simulink model "three_phase_power_meter_iec"  (R2026a)
settings: Solver=VariableStepAuto
undefined symbols (not defined in the file): glb_time, grid_emu, magnitude
libraries: simulink x12
(part 1 of 3)
settings Model: Creator=dbagn  LastModifiedBy=dbagn

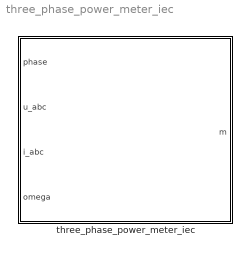
== system three_phase_power_meter_iec ==
  three_phase_power_meter_iec : Subsystem  mask{period=pi/grid_emu.omega_grid_nom, ts=glb_time.ts_afe, enable_time=0.025}
      mask prompts: period "period (s)"; ts "sampling time (s)"; enable_time "enable_time (s)"

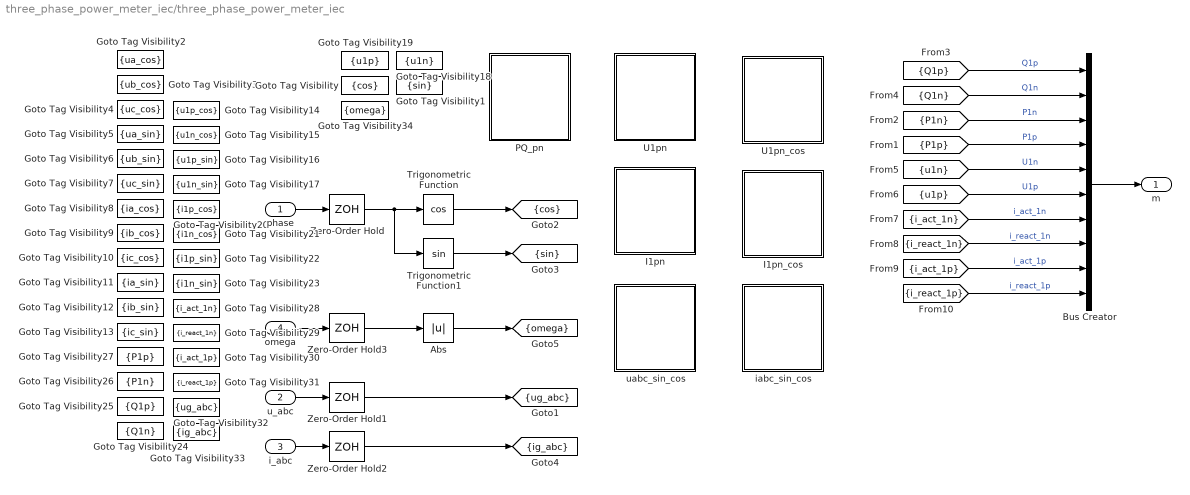
== system three_phase_power_meter_iec/three_phase_power_meter_iec ==
  phase : Inport
  u_abc : Inport  Port=2
  i_abc : Inport  Port=3
  omega : Inport  Port=4
  Abs : Abs  SaturateOnIntegerOverflow=off
  Bus Creator : BusCreator  Inputs=10
  Goto Tag Visibility : GotoTagVisibility  GotoTag=cos
  Goto Tag Visibility1 : GotoTagVisibility  GotoTag=sin
  Goto Tag Visibility10 : GotoTagVisibility  GotoTag=ic_cos
  Goto Tag Visibility11 : GotoTagVisibility  GotoTag=ia_sin
  Goto Tag Visibility12 : GotoTagVisibility  GotoTag=ib_sin
  Goto Tag Visibility13 : GotoTagVisibility  GotoTag=ic_sin
  Goto Tag Visibility14 : GotoTagVisibility  GotoTag=u1p_cos
  Goto Tag Visibility15 : GotoTagVisibility  GotoTag=u1n_cos
  Goto Tag Visibility16 : GotoTagVisibility  GotoTag=u1p_sin
  Goto Tag Visibility17 : GotoTagVisibility  GotoTag=u1n_sin
  Goto Tag Visibility18 : GotoTagVisibility  GotoTag=u1n
  Goto Tag Visibility19 : GotoTagVisibility  GotoTag=u1p
  Goto Tag Visibility2 : GotoTagVisibility  GotoTag=ua_cos
  Goto Tag Visibility20 : GotoTagVisibility  GotoTag=i1p_cos
  Goto Tag Visibility21 : GotoTagVisibility  GotoTag=i1n_cos
  Goto Tag Visibility22 : GotoTagVisibility  GotoTag=i1p_sin
  Goto Tag Visibility23 : GotoTagVisibility  GotoTag=i1n_sin
  Goto Tag Visibility24 : GotoTagVisibility  GotoTag=Q1n
  Goto Tag Visibility25 : GotoTagVisibility  GotoTag=Q1p
  Goto Tag Visibility26 : GotoTagVisibility  GotoTag=P1n
  Goto Tag Visibility27 : GotoTagVisibility  GotoTag=P1p
  Goto Tag Visibility28 : GotoTagVisibility  GotoTag=i_act_1n
  Goto Tag Visibility29 : GotoTagVisibility  GotoTag=i_react_1n
  Goto Tag Visibility3 : GotoTagVisibility  GotoTag=ub_cos
  Goto Tag Visibility30 : GotoTagVisibility  GotoTag=i_act_1p
  Goto Tag Visibility31 : GotoTagVisibility  GotoTag=i_react_1p
  Goto Tag Visibility32 : GotoTagVisibility  GotoTag=ug_abc
  Goto Tag Visibility33 : GotoTagVisibility  GotoTag=ig_abc
  Goto Tag Visibility34 : GotoTagVisibility  GotoTag=omega
  Goto Tag Visibility4 : GotoTagVisibility  GotoTag=uc_cos
  Goto Tag Visibility5 : GotoTagVisibility  GotoTag=ua_sin
  Goto Tag Visibility6 : GotoTagVisibility  GotoTag=ub_sin
  Goto Tag Visibility7 : GotoTagVisibility  GotoTag=uc_sin
  Goto Tag Visibility8 : GotoTagVisibility  GotoTag=ia_cos
  Goto Tag Visibility9 : GotoTagVisibility  GotoTag=ib_cos
  I1pn : Subsystem
  I1pn_cos : Subsystem
  PQ_pn : Subsystem
  Trigonometric Function : Trigonometry  Operator=cos
  Trigonometric Function1 : Trigonometry
  U1pn : Subsystem
  U1pn_cos : Subsystem
  Zero-Order Hold{,1..3} (4 alike) : ZeroOrderHold  SampleTime=ts
  iabc_sin_cos : Subsystem
  uabc_sin_cos : Subsystem
  m : Outport
  tag scope: cos=scoped, ig_abc=scoped, omega=scoped, sin=scoped, ug_abc=scoped
  wires:
  Abs/1 -> [omega]
  [Q1p] -> Bus Creator/1  "Q1p"
  [Q1n] -> Bus Creator/2  "Q1n"
  [P1n] -> Bus Creator/3  "P1n"
  [P1p] -> Bus Creator/4  "P1p"
  Zero-Order Hold3/1 -> Abs/1
  omega/1 -> Zero-Order Hold3/1
  Zero-Order Hold1/1 -> [ug_abc]
  Zero-Order Hold2/1 -> [ig_abc]
  Zero-Order Hold/1 -> Trigonometric Function1/1, Trigonometric Function/1
  Bus Creator/1 -> m/1
  i_abc/1 -> Zero-Order Hold2/1
  u_abc/1 -> Zero-Order Hold1/1
  [i_react_1p] -> Bus Creator/10  "i_react_1p"
  [i_act_1p] -> Bus Creator/9  "i_act_1p"
  [i_react_1n] -> Bus Creator/8  "i_react_1n"
  [i_act_1n] -> Bus Creator/7  "i_act_1n"
  [u1p] -> Bus Creator/6  "U1p"
  [u1n] -> Bus Creator/5  "U1n"
  phase/1 -> Zero-Order Hold/1
  Trigonometric Function/1 -> [cos]
  Trigonometric Function1/1 -> [sin]

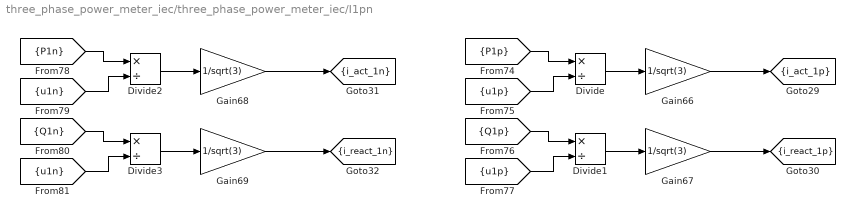
== system three_phase_power_meter_iec/three_phase_power_meter_iec/I1pn ==
  Divide{,1..3} (4 alike) : Product  Inputs=*/
  Gain{66..69} (4 alike) : Gain  Gain=1/sqrt(3)
  tag scope: i_act_1n=scoped, i_act_1p=scoped, i_react_1n=scoped, i_react_1p=scoped
  wires:
  [P1n] -> Divide2/1
  [Q1n] -> Divide3/1
  [u1n] -> Divide3/2
  [Q1p] -> Divide1/1
  Gain69/1 -> [i_react_1n]
  [u1p] -> Divide/2
  Divide/1 -> Gain66/1
  Divide3/1 -> Gain69/1
  Divide1/1 -> Gain67/1
  Gain66/1 -> [i_act_1p]
  [u1n] -> Divide2/2
  Gain67/1 -> [i_react_1p]
  [u1p] -> Divide1/2
  Gain68/1 -> [i_act_1n]
  Divide2/1 -> Gain68/1
  [P1p] -> Divide/1

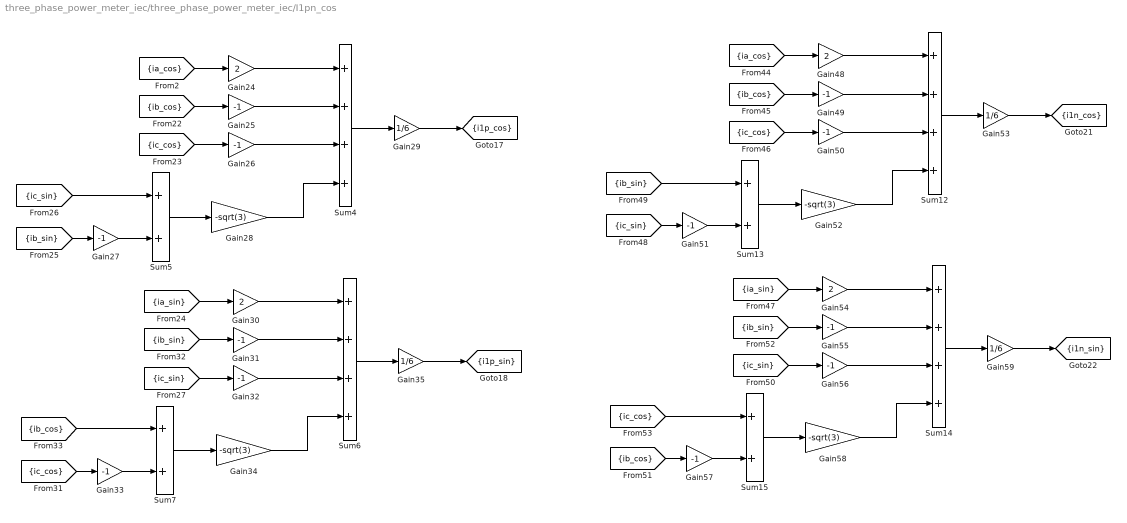
== system three_phase_power_meter_iec/three_phase_power_meter_iec/I1pn_cos ==
  Gain{24,30,48,54} (4 alike) : Gain  Gain=2
  Gain{25..27,31..33,49..51,55..57} (12 alike) : Gain  Gain=-1
  Gain{28,34,52,58} (4 alike) : Gain  Gain=-sqrt(3)
  Gain{29,35,53,59} (4 alike) : Gain  Gain=1/6
  Sum{4,6,12,14} (4 alike) : Sum  Inputs=++++
  Sum{5,7,13,15} (4 alike) : Sum
  tag scope: i1n_cos=scoped, i1n_sin=scoped, i1p_cos=scoped, i1p_sin=scoped
  wires:
  Gain57/1 -> Sum15/2
  [ib_cos] -> Gain25/1
  Sum15/1 -> Gain58/1
  Gain50/1 -> Sum12/3
  [ib_sin] -> Gain31/1
  Gain56/1 -> Sum14/3
  [ic_cos] -> Gain50/1
  Gain48/1 -> Sum12/1
  [ia_sin] -> Gain30/1
  Gain51/1 -> Sum13/2
  Sum6/1 -> Gain35/1
  Gain59/1 -> [i1n_sin]
  Gain58/1 -> Sum14/4
  Gain26/1 -> Sum4/3
  [ib_sin] -> Gain55/1
  Gain32/1 -> Sum6/3
  Gain28/1 -> Sum4/4
  [ia_cos] -> Gain24/1
  Gain34/1 -> Sum6/4
  [ic_cos] -> Sum15/1
  [ib_cos] -> Gain57/1
  Gain33/1 -> Sum7/2
  Sum5/1 -> Gain28/1
  Sum7/1 -> Gain34/1
  Gain53/1 -> [i1n_cos]
  [ib_sin] -> Gain27/1
  Gain25/1 -> Sum4/2
  [ic_sin] -> Gain56/1
  [ib_sin] -> Sum13/1
  [ib_cos] -> Gain49/1
  Gain24/1 -> Sum4/1
  Sum4/1 -> Gain29/1
  Sum13/1 -> Gain52/1
  [ia_sin] -> Gain54/1
  [ia_cos] -> Gain48/1
  [ic_cos] -> Gain26/1
  Gain30/1 -> Sum6/1
  [ic_sin] -> Sum5/1
  Gain55/1 -> Sum14/2
  [ic_cos] -> Gain33/1
  [ic_sin] -> Gain32/1
  Gain29/1 -> [i1p_cos]
  [ic_sin] -> Gain51/1
  Sum14/1 -> Gain59/1
  Gain31/1 -> Sum6/2
  Gain52/1 -> Sum12/4
  [ib_cos] -> Sum7/1
  Gain54/1 -> Sum14/1
  Gain49/1 -> Sum12/2
  Gain27/1 -> Sum5/2
  Sum12/1 -> Gain53/1
  Gain35/1 -> [i1p_sin]

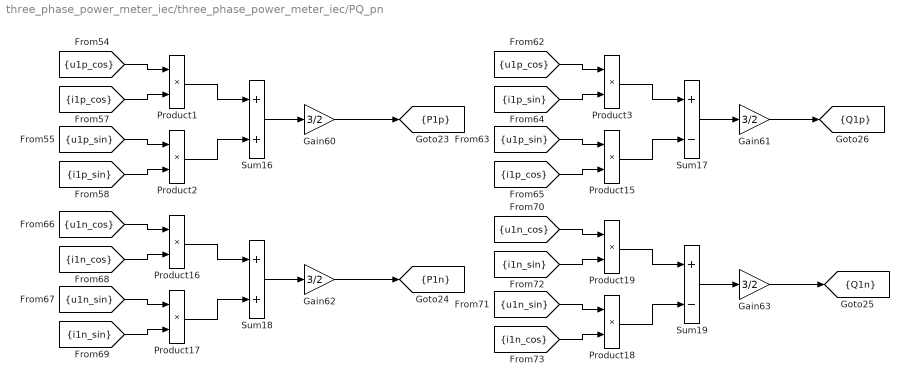
== system three_phase_power_meter_iec/three_phase_power_meter_iec/PQ_pn ==
  Gain{60..63} (4 alike) : Gain  Gain=3/2
  Product{1..3,15..19} (8 alike) : Product  RndMeth=Zero
  Sum16 : Sum
  Sum17 : Sum  Inputs=+-
  Sum18 : Sum
  Sum19 : Sum  Inputs=+-
  tag scope: P1n=scoped, P1p=scoped, Q1n=scoped, Q1p=scoped
  wires:
  Product3/1 -> Sum17/1
  [i1n_sin] -> Product19/2
  Sum16/1 -> Gain60/1
  [u1n_cos] -> Product16/1
  [u1n_sin] -> Product18/1
  [u1n_sin] -> Product17/1
  [u1p_cos] -> Product3/1
  [u1p_sin] -> Product2/1
  [i1p_sin] -> Product3/2
  Product15/1 -> Sum17/2
  [u1p_sin] -> Product15/1
  [i1p_cos] -> Product15/2
  Product2/1 -> Sum16/2
  Gain61/1 -> [Q1p]
  Sum18/1 -> Gain62/1
  Gain62/1 -> [P1n]
  [i1p_cos] -> Product1/2
  Sum17/1 -> Gain61/1
  Product1/1 -> Sum16/1
  [u1p_cos] -> Product1/1
  Product18/1 -> Sum19/2
  Product17/1 -> Sum18/2
  Gain63/1 -> [Q1n]
  Product16/1 -> Sum18/1
  [i1n_cos] -> Product18/2
  [i1n_cos] -> Product16/2
  [u1n_cos] -> Product19/1
  Sum19/1 -> Gain63/1
  Gain60/1 -> [P1p]
  Product19/1 -> Sum19/1
  [i1n_sin] -> Product17/2
  [i1p_sin] -> Product2/2

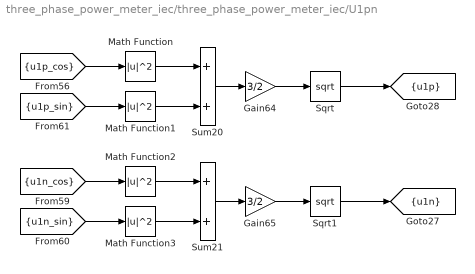
== system three_phase_power_meter_iec/three_phase_power_meter_iec/U1pn ==
  Gain64 : Gain  Gain=3/2
  Gain65 : Gain  Gain=3/2
  Math Function{,1..3} (4 alike) : Math  Operator=magnitude^2  SignedPower=on
  Sqrt : Sqrt
  Sqrt1 : Sqrt
  Sum20 : Sum
  Sum21 : Sum
  tag scope: u1n=scoped, u1p=scoped
  wires:
  [u1p_sin] -> Math Function1/1
  Gain65/1 -> Sqrt1/1
  [u1n_cos] -> Math Function2/1
  Math Function/1 -> Sum20/1
  [u1n_sin] -> Math Function3/1
  Sum21/1 -> Gain65/1
  Sqrt/1 -> [u1p]
  Gain64/1 -> Sqrt/1
  Sqrt1/1 -> [u1n]
  Math Function2/1 -> Sum21/1
  Math Function1/1 -> Sum20/2
  [u1p_cos] -> Math Function/1
  Math Function3/1 -> Sum21/2
  Sum20/1 -> Gain64/1

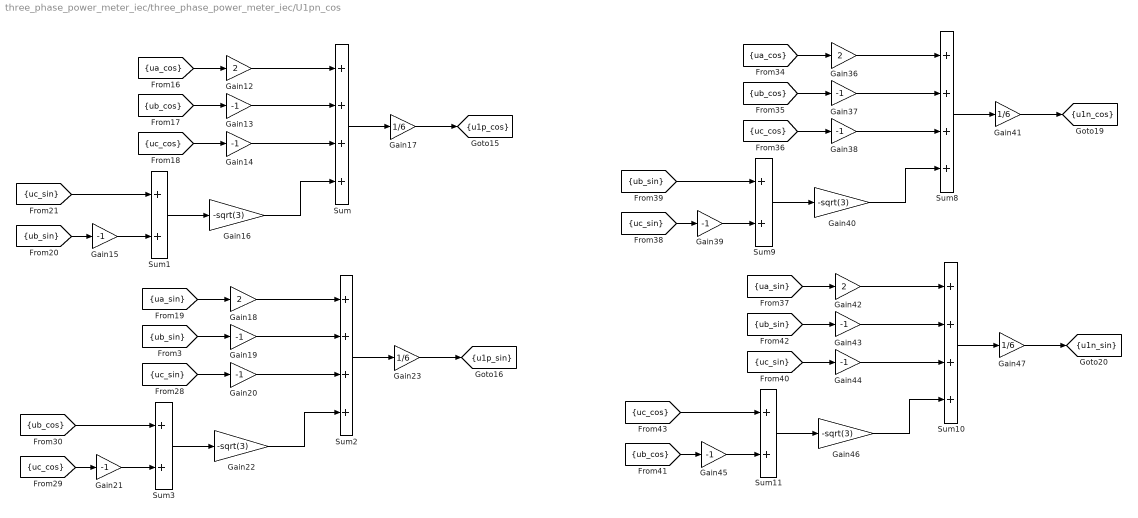
== system three_phase_power_meter_iec/three_phase_power_meter_iec/U1pn_cos ==
  Gain{12,18,36,42} (4 alike) : Gain  Gain=2
  Gain{13..15,19..21,37..39,43..45} (12 alike) : Gain  Gain=-1
  Gain{16,22,40,46} (4 alike) : Gain  Gain=-sqrt(3)
  Gain{17,23,41,47} (4 alike) : Gain  Gain=1/6
  Sum{,2,8,10} (4 alike) : Sum  Inputs=++++
  Sum{1,3,9,11} (4 alike) : Sum
  tag scope: u1n_cos=scoped, u1n_sin=scoped, u1p_cos=scoped, u1p_sin=scoped
  wires:
  Gain12/1 -> Sum/1
  [ua_sin] -> Gain18/1
  Sum9/1 -> Gain40/1
  [uc_cos] -> Sum11/1
  Gain18/1 -> Sum2/1
  [ub_sin] -> Gain19/1
  Gain45/1 -> Sum11/2
  Sum2/1 -> Gain23/1
  Gain19/1 -> Sum2/2
  Gain22/1 -> Sum2/4
  Gain46/1 -> Sum10/4
  Gain47/1 -> [u1n_sin]
  Sum10/1 -> Gain47/1
  Gain17/1 -> [u1p_cos]
  [uc_cos] -> Gain21/1
  [uc_cos] -> Gain14/1
  Gain38/1 -> Sum8/3
  Gain23/1 -> [u1p_sin]
  [uc_sin] -> Gain39/1
  [ua_sin] -> Gain42/1
  Sum1/1 -> Gain16/1
  [ub_sin] -> Gain43/1
  [ub_sin] -> Gain15/1
  [ub_cos] -> Gain13/1
  Gain44/1 -> Sum10/3
  Gain20/1 -> Sum2/3
  Gain37/1 -> Sum8/2
  [uc_sin] -> Sum1/1
  Gain16/1 -> Sum/4
  Gain41/1 -> [u1n_cos]
  Gain21/1 -> Sum3/2
  [uc_cos] -> Gain38/1
  Sum/1 -> Gain17/1
  Gain43/1 -> Sum10/2
  Gain14/1 -> Sum/3
  Gain42/1 -> Sum10/1
  [uc_sin] -> Gain44/1
  [ub_cos] -> Sum3/1
  [ua_cos] -> Gain12/1
  Gain39/1 -> Sum9/2
  [uc_sin] -> Gain20/1
  Sum11/1 -> Gain46/1
  Sum8/1 -> Gain41/1
  [ub_sin] -> Sum9/1
  Gain36/1 -> Sum8/1
  Gain40/1 -> Sum8/4
  Sum3/1 -> Gain22/1
  [ua_cos] -> Gain36/1
  Gain13/1 -> Sum/2
  [ub_cos] -> Gain37/1
  [ub_cos] -> Gain45/1
  Gain15/1 -> Sum1/2

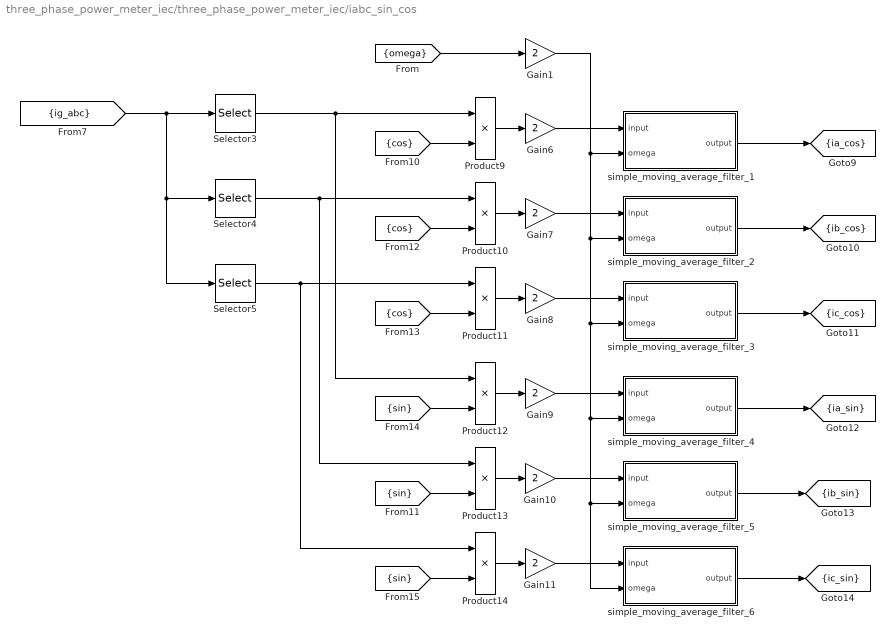
== system three_phase_power_meter_iec/three_phase_power_meter_iec/iabc_sin_cos ==
  Gain{1,6..11} (7 alike) : Gain  Gain=2
  Product{9..14} (6 alike) : Product  RndMeth=Zero
  Selector3 : Selector  InputPortWidth=3  IndexOptions=Index vector (dialog)  Indices=1  OutputSizes=1
  Selector4 : Selector  InputPortWidth=3  IndexOptions=Index vector (dialog)  Indices=2  OutputSizes=1
  Selector5 : Selector  InputPortWidth=3  IndexOptions=Index vector (dialog)  Indices=3  OutputSizes=1
  simple_moving_average_filter_1 : Subsystem
  simple_moving_average_filter_2 : Subsystem
  simple_moving_average_filter_3 : Subsystem
  simple_moving_average_filter_4 : Subsystem
  simple_moving_average_filter_5 : Subsystem
  simple_moving_average_filter_6 : Subsystem
  tag scope: ia_cos=scoped, ia_sin=scoped, ib_cos=scoped, ib_sin=scoped, ic_cos=scoped, ic_sin=scoped
  wires:
  Gain1/1 -> simple_moving_average_filter_1/2(omega), simple_moving_average_filter_2/2(omega), simple_moving_average_filter_3/2(omega), simple_moving_average_filter_4/2(omega), simple_moving_average_filter_6/2(omega), simple_moving_average_filter_5/2(omega)
  [omega] -> Gain1/1
  simple_moving_average_filter_1/1(output) -> [ia_cos]
  Gain6/1 -> simple_moving_average_filter_1/1(input)
  simple_moving_average_filter_5/1(output) -> [ib_sin]
  simple_moving_average_filter_3/1(output) -> [ic_cos]
  simple_moving_average_filter_4/1(output) -> [ia_sin]
  simple_moving_average_filter_6/1(output) -> [ic_sin]
  simple_moving_average_filter_2/1(output) -> [ib_cos]
  Product14/1 -> Gain11/1
  [sin] -> Product12/2
  Gain11/1 -> simple_moving_average_filter_6/1(input)
  Selector4/1 -> Product13/1, Product10/1
  [sin] -> Product14/2
  Product9/1 -> Gain6/1
  Product10/1 -> Gain7/1
  Gain10/1 -> simple_moving_average_filter_5/1(input)
  Selector3/1 -> Product12/1, Product9/1
  Gain7/1 -> simple_moving_average_filter_2/1(input)
  [cos] -> Product10/2
  [cos] -> Product9/2
  Gain9/1 -> simple_moving_average_filter_4/1(input)
  Product11/1 -> Gain8/1
  [sin] -> Product13/2
  [ig_abc] -> Selector5/1, Selector4/1, Selector3/1
  [cos] -> Product11/2
  Gain8/1 -> simple_moving_average_filter_3/1(input)
  Product12/1 -> Gain9/1
  Product13/1 -> Gain10/1
  Selector5/1 -> Product14/1, Product11/1

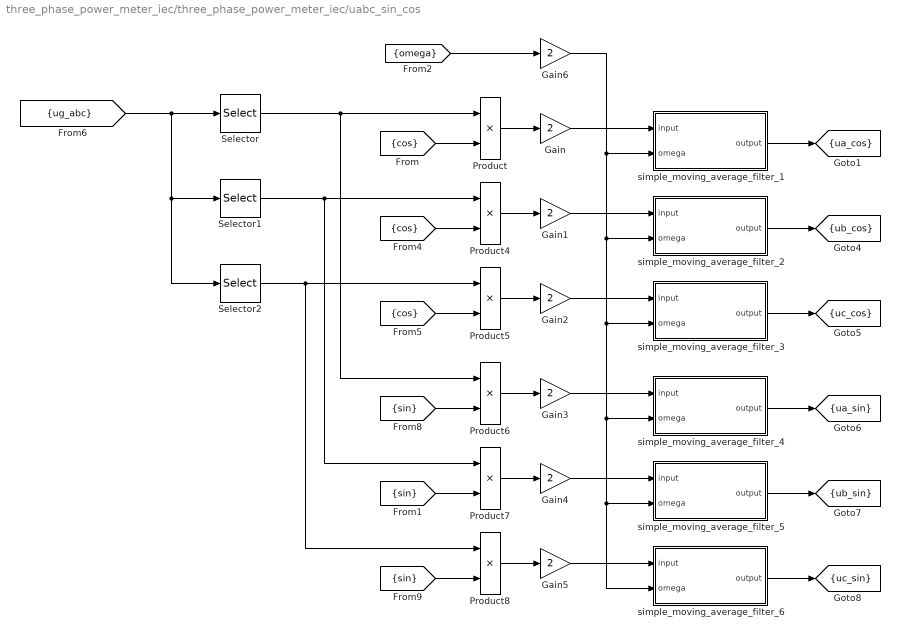
== system three_phase_power_meter_iec/three_phase_power_meter_iec/uabc_sin_cos ==
  Gain{,1..6} (7 alike) : Gain  Gain=2
  Product{,4..8} (6 alike) : Product  RndMeth=Zero
  Selector : Selector  InputPortWidth=3  IndexOptions=Index vector (dialog)  Indices=1  OutputSizes=1
  Selector1 : Selector  InputPortWidth=3  IndexOptions=Index vector (dialog)  Indices=2  OutputSizes=1
  Selector2 : Selector  InputPortWidth=3  IndexOptions=Index vector (dialog)  Indices=3  OutputSizes=1
  simple_moving_average_filter_1 : Subsystem
  simple_moving_average_filter_2 : Subsystem
  simple_moving_average_filter_3 : Subsystem
  simple_moving_average_filter_4 : Subsystem
  simple_moving_average_filter_5 : Subsystem
  simple_moving_average_filter_6 : Subsystem
  tag scope: ua_cos=scoped, ua_sin=scoped, ub_cos=scoped, ub_sin=scoped, uc_cos=scoped, uc_sin=scoped
  wires:
  [omega] -> Gain6/1
  Gain6/1 -> simple_moving_average_filter_2/2(omega), simple_moving_average_filter_3/2(omega), simple_moving_average_filter_4/2(omega), simple_moving_average_filter_6/2(omega), simple_moving_average_filter_5/2(omega), simple_moving_average_filter_1/2(omega)
  simple_moving_average_filter_6/1(output) -> [uc_sin]
  simple_moving_average_filter_5/1(output) -> [ub_sin]
  simple_moving_average_filter_4/1(output) -> [ua_sin]
  simple_moving_average_filter_3/1(output) -> [uc_cos]
  simple_moving_average_filter_2/1(output) -> [ub_cos]
  simple_moving_average_filter_1/1(output) -> [ua_cos]
  Selector2/1 -> Product5/1, Product8/1
  [cos] -> Product/2
  [sin] -> Product6/2
  Product8/1 -> Gain5/1
  [cos] -> Product5/2
  Product6/1 -> Gain3/1
  [sin] -> Product7/2
  Selector1/1 -> Product4/1, Product7/1
  Gain4/1 -> simple_moving_average_filter_5/1(input)
  Product7/1 -> Gain4/1
  Selector/1 -> Product/1, Product6/1
  Product4/1 -> Gain1/1
  [sin] -> Product8/2
  Gain/1 -> simple_moving_average_filter_1/1(input)
  Gain2/1 -> simple_moving_average_filter_3/1(input)
  Gain3/1 -> simple_moving_average_filter_4/1(input)
  Product5/1 -> Gain2/1
  [ug_abc] -> Selector/1, Selector1/1, Selector2/1
  Gain5/1 -> simple_moving_average_filter_6/1(input)
  [cos] -> Product4/2
  Gain1/1 -> simple_moving_average_filter_2/1(input)
  Product/1 -> Gain/1

== system three_phase_power_meter_iec/three_phase_power_meter_iec/iabc_sin_cos/simple_moving_average_filter_1 ==
  input : Inport
  omega : Inport  Port=2
  dmavg_flt : Subsystem  mask{ts=ts, enable_time=enable_time}
      mask prompts: ts "sampling time (s)"; enable_time "enable_time (s)"
      mask Display:
      | disp('dmavg_flt()');
      | port_label('input', 1, 'input');
      | port_label('input', 2, 'omega');
      | port_label('output', 1, 'output');
  output : Outport
  wires:
  dmavg_flt/1(output) -> output/1
  omega/1 -> dmavg_flt/2(omega)
  input/1 -> dmavg_flt/1(input)

== system three_phase_power_meter_iec/three_phase_power_meter_iec/iabc_sin_cos/simple_moving_average_filter_2 ==
  input : Inport
  omega : Inport  Port=2
  dmavg_flt : Subsystem  mask{ts=ts, enable_time=enable_time}
      mask prompts: ts "sampling time (s)"; enable_time "enable_time (s)"
      mask Display:
      | disp('dmavg_flt()');
      | port_label('input', 1, 'input');
      | port_label('input', 2, 'omega');
      | port_label('output', 1, 'output');
  output : Outport
  wires:
  input/1 -> dmavg_flt/1(input)
  omega/1 -> dmavg_flt/2(omega)
  dmavg_flt/1(output) -> output/1

== system three_phase_power_meter_iec/three_phase_power_meter_iec/iabc_sin_cos/simple_moving_average_filter_3 ==
  input : Inport
  omega : Inport  Port=2
  dmavg_flt : Subsystem  mask{ts=ts, enable_time=enable_time}
      mask prompts: ts "sampling time (s)"; enable_time "enable_time (s)"
      mask Display:
      | disp('dmavg_flt()');
      | port_label('input', 1, 'input');
      | port_label('input', 2, 'omega');
      | port_label('output', 1, 'output');
  output : Outport
  wires:
  dmavg_flt/1(output) -> output/1
  omega/1 -> dmavg_flt/2(omega)
  input/1 -> dmavg_flt/1(input)

== system three_phase_power_meter_iec/three_phase_power_meter_iec/iabc_sin_cos/simple_moving_average_filter_4 ==
  input : Inport
  omega : Inport  Port=2
  dmavg_flt : Subsystem  mask{ts=ts, enable_time=enable_time}
      mask prompts: ts "sampling time (s)"; enable_time "enable_time (s)"
      mask Display:
      | disp('dmavg_flt()');
      | port_label('input', 1, 'input');
      | port_label('input', 2, 'omega');
      | port_label('output', 1, 'output');
  output : Outport
  wires:
  input/1 -> dmavg_flt/1(input)
  omega/1 -> dmavg_flt/2(omega)
  dmavg_flt/1(output) -> output/1

== system three_phase_power_meter_iec/three_phase_power_meter_iec/iabc_sin_cos/simple_moving_average_filter_5 ==
  input : Inport
  omega : Inport  Port=2
  dmavg_flt : Subsystem  mask{ts=ts, enable_time=enable_time}
      mask prompts: ts "sampling time (s)"; enable_time "enable_time (s)"
      mask Display:
      | disp('dmavg_flt()');
      | port_label('input', 1, 'input');
      | port_label('input', 2, 'omega');
      | port_label('output', 1, 'output');
  output : Outport
  wires:
  dmavg_flt/1(output) -> output/1
  omega/1 -> dmavg_flt/2(omega)
  input/1 -> dmavg_flt/1(input)

== system three_phase_power_meter_iec/three_phase_power_meter_iec/iabc_sin_cos/simple_moving_average_filter_6 ==
  input : Inport
  omega : Inport  Port=2
  dmavg_flt : Subsystem  mask{ts=ts, enable_time=enable_time}
      mask prompts: ts "sampling time (s)"; enable_time "enable_time (s)"
      mask Display:
      | disp('dmavg_flt()');
      | port_label('input', 1, 'input');
      | port_label('input', 2, 'omega');
      | port_label('output', 1, 'output');
  output : Outport
  wires:
  input/1 -> dmavg_flt/1(input)
  omega/1 -> dmavg_flt/2(omega)
  dmavg_flt/1(output) -> output/1

== system three_phase_power_meter_iec/three_phase_power_meter_iec/uabc_sin_cos/simple_moving_average_filter_1 ==
  input : Inport
  omega : Inport  Port=2
  dmavg_flt : Subsystem  mask{ts=ts, enable_time=enable_time}
      mask prompts: ts "sampling time (s)"; enable_time "enable_time (s)"
      mask Display:
      | disp('dmavg_flt()');
      | port_label('input', 1, 'input');
      | port_label('input', 2, 'omega');
      | port_label('output', 1, 'output');
  output : Outport
  wires:
  dmavg_flt/1(output) -> output/1
  omega/1 -> dmavg_flt/2(omega)
  input/1 -> dmavg_flt/1(input)

== system three_phase_power_meter_iec/three_phase_power_meter_iec/uabc_sin_cos/simple_moving_average_filter_2 ==
  input : Inport
  omega : Inport  Port=2
  dmavg_flt : Subsystem  mask{ts=ts, enable_time=enable_time}
      mask prompts: ts "sampling time (s)"; enable_time "enable_time (s)"
      mask Display:
      | disp('dmavg_flt()');
      | port_label('input', 1, 'input');
      | port_label('input', 2, 'omega');
      | port_label('output', 1, 'output');
  output : Outport
  wires:
  input/1 -> dmavg_flt/1(input)
  omega/1 -> dmavg_flt/2(omega)
  dmavg_flt/1(output) -> output/1

== system three_phase_power_meter_iec/three_phase_power_meter_iec/uabc_sin_cos/simple_moving_average_filter_3 ==
  input : Inport
  omega : Inport  Port=2
  dmavg_flt : Subsystem  mask{ts=ts, enable_time=enable_time}
      mask prompts: ts "sampling time (s)"; enable_time "enable_time (s)"
      mask Display:
      | disp('dmavg_flt()');
      | port_label('input', 1, 'input');
      | port_label('input', 2, 'omega');
      | port_label('output', 1, 'output');
  output : Outport
  wires:
  dmavg_flt/1(output) -> output/1
  omega/1 -> dmavg_flt/2(omega)
  input/1 -> dmavg_flt/1(input)

== system three_phase_power_meter_iec/three_phase_power_meter_iec/uabc_sin_cos/simple_moving_average_filter_4 ==
  input : Inport
  omega : Inport  Port=2
  dmavg_flt : Subsystem  mask{ts=ts, enable_time=enable_time}
      mask prompts: ts "sampling time (s)"; enable_time "enable_time (s)"
      mask Display:
      | disp('dmavg_flt()');
      | port_label('input', 1, 'input');
      | port_label('input', 2, 'omega');
      | port_label('output', 1, 'output');
  output : Outport
  wires:
  input/1 -> dmavg_flt/1(input)
  omega/1 -> dmavg_flt/2(omega)
  dmavg_flt/1(output) -> output/1

== system three_phase_power_meter_iec/three_phase_power_meter_iec/uabc_sin_cos/simple_moving_average_filter_5 ==
  input : Inport
  omega : Inport  Port=2
  dmavg_flt : Subsystem  mask{ts=ts, enable_time=enable_time}
      mask prompts: ts "sampling time (s)"; enable_time "enable_time (s)"
      mask Display:
      | disp('dmavg_flt()');
      | port_label('input', 1, 'input');
      | port_label('input', 2, 'omega');
      | port_label('output', 1, 'output');
  output : Outport
  wires:
  dmavg_flt/1(output) -> output/1
  omega/1 -> dmavg_flt/2(omega)
  input/1 -> dmavg_flt/1(input)

== system three_phase_power_meter_iec/three_phase_power_meter_iec/uabc_sin_cos/simple_moving_average_filter_6 ==
  input : Inport
  omega : Inport  Port=2
  dmavg_flt : Subsystem  mask{ts=ts, enable_time=enable_time}
      mask prompts: ts "sampling time (s)"; enable_time "enable_time (s)"
      mask Display:
      | disp('dmavg_flt()');
      | port_label('input', 1, 'input');
      | port_label('input', 2, 'omega');
      | port_label('output', 1, 'output');
  output : Outport
  wires:
  input/1 -> dmavg_flt/1(input)
  omega/1 -> dmavg_flt/2(omega)
  dmavg_flt/1(output) -> output/1

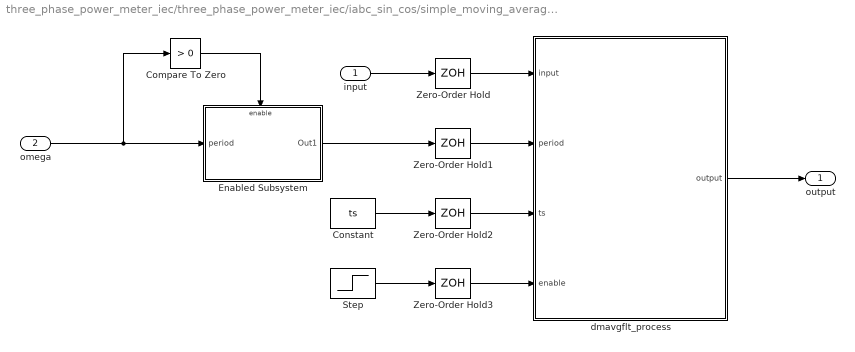
== system three_phase_power_meter_iec/three_phase_power_meter_iec/iabc_sin_cos/simple_moving_average_filter_1/dmavg_flt ==
  input : Inport
  omega : Inport  Port=2
  Compare To Zero : simulink/Logic and Bit Operations/Compare To Zero  relop=>  OutDataTypeStr=boolean
  Constant : Constant  Value=ts
  Enabled Subsystem : Subsystem  TreatAsAtomicUnit=on
  Step : Step  Time=enable_time
  Zero-Order Hold{,1..3} (4 alike) : ZeroOrderHold  SampleTime=-1
  dmavgflt_process : MATLAB Function  TreatAsAtomicUnit=on
  output : Outport
  wires:
  Zero-Order Hold3/1 -> dmavgflt_process/4(enable)
  Step/1 -> Zero-Order Hold3/1
  Zero-Order Hold1/1 -> dmavgflt_process/2(period)
  Zero-Order Hold2/1 -> dmavgflt_process/3(ts)
  Constant/1 -> Zero-Order Hold2/1
  Enabled Subsystem/1(Out1) -> Zero-Order Hold1/1
  Zero-Order Hold/1 -> dmavgflt_process/1(input)
  input/1 -> Zero-Order Hold/1
  omega/1 -> Enabled Subsystem/1(period), Compare To Zero/1
  Compare To Zero/1 -> Enabled Subsystem/Enable
  dmavgflt_process/1(output) -> output/1

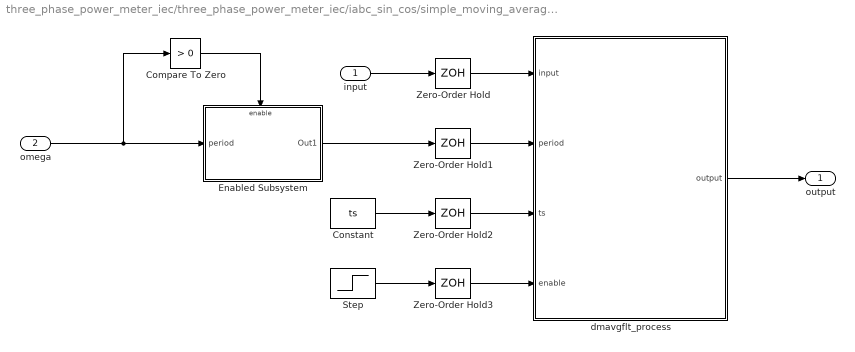
== system three_phase_power_meter_iec/three_phase_power_meter_iec/iabc_sin_cos/simple_moving_average_filter_2/dmavg_flt ==
  input : Inport
  omega : Inport  Port=2
  Compare To Zero : simulink/Logic and Bit Operations/Compare To Zero  relop=>  OutDataTypeStr=boolean
  Constant : Constant  Value=ts
  Enabled Subsystem : Subsystem  TreatAsAtomicUnit=on
  Step : Step  Time=enable_time
  Zero-Order Hold{,1..3} (4 alike) : ZeroOrderHold  SampleTime=-1
  dmavgflt_process : MATLAB Function  TreatAsAtomicUnit=on
  output : Outport
  wires:
  dmavgflt_process/1(output) -> output/1
  Compare To Zero/1 -> Enabled Subsystem/Enable
  omega/1 -> Compare To Zero/1, Enabled Subsystem/1(period)
  input/1 -> Zero-Order Hold/1
  Zero-Order Hold/1 -> dmavgflt_process/1(input)
  Enabled Subsystem/1(Out1) -> Zero-Order Hold1/1
  Constant/1 -> Zero-Order Hold2/1
  Zero-Order Hold2/1 -> dmavgflt_process/3(ts)
  Zero-Order Hold1/1 -> dmavgflt_process/2(period)
  Step/1 -> Zero-Order Hold3/1
  Zero-Order Hold3/1 -> dmavgflt_process/4(enable)

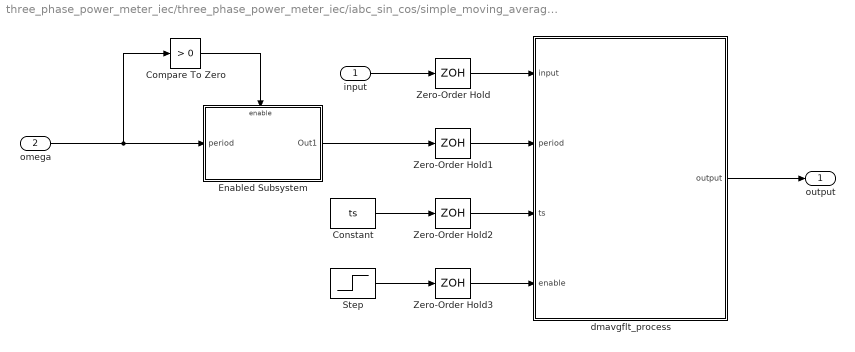
== system three_phase_power_meter_iec/three_phase_power_meter_iec/iabc_sin_cos/simple_moving_average_filter_3/dmavg_flt ==
  input : Inport
  omega : Inport  Port=2
  Compare To Zero : simulink/Logic and Bit Operations/Compare To Zero  relop=>  OutDataTypeStr=boolean
  Constant : Constant  Value=ts
  Enabled Subsystem : Subsystem  TreatAsAtomicUnit=on
  Step : Step  Time=enable_time
  Zero-Order Hold{,1..3} (4 alike) : ZeroOrderHold  SampleTime=-1
  dmavgflt_process : MATLAB Function  TreatAsAtomicUnit=on
  output : Outport
  wires:
  Zero-Order Hold3/1 -> dmavgflt_process/4(enable)
  Step/1 -> Zero-Order Hold3/1
  Zero-Order Hold1/1 -> dmavgflt_process/2(period)
  Zero-Order Hold2/1 -> dmavgflt_process/3(ts)
  Constant/1 -> Zero-Order Hold2/1
  Enabled Subsystem/1(Out1) -> Zero-Order Hold1/1
  Zero-Order Hold/1 -> dmavgflt_process/1(input)
  input/1 -> Zero-Order Hold/1
  omega/1 -> Enabled Subsystem/1(period), Compare To Zero/1
  Compare To Zero/1 -> Enabled Subsystem/Enable
  dmavgflt_process/1(output) -> output/1

== system three_phase_power_meter_iec/three_phase_power_meter_iec/iabc_sin_cos/simple_moving_average_filter_4/dmavg_flt ==
  input : Inport
  omega : Inport  Port=2
  Compare To Zero : simulink/Logic and Bit Operations/Compare To Zero  relop=>  OutDataTypeStr=boolean
  Constant : Constant  Value=ts
  Enabled Subsystem : Subsystem  TreatAsAtomicUnit=on
  Step : Step  Time=enable_time
  Zero-Order Hold{,1..3} (4 alike) : ZeroOrderHold  SampleTime=-1
  dmavgflt_process : MATLAB Function  TreatAsAtomicUnit=on
  output : Outport
  wires:
  dmavgflt_process/1(output) -> output/1
  Compare To Zero/1 -> Enabled Subsystem/Enable
  omega/1 -> Compare To Zero/1, Enabled Subsystem/1(period)
  input/1 -> Zero-Order Hold/1
  Zero-Order Hold/1 -> dmavgflt_process/1(input)
  Enabled Subsystem/1(Out1) -> Zero-Order Hold1/1
  Constant/1 -> Zero-Order Hold2/1
  Zero-Order Hold2/1 -> dmavgflt_process/3(ts)
  Zero-Order Hold1/1 -> dmavgflt_process/2(period)
  Step/1 -> Zero-Order Hold3/1
  Zero-Order Hold3/1 -> dmavgflt_process/4(enable)

== system three_phase_power_meter_iec/three_phase_power_meter_iec/iabc_sin_cos/simple_moving_average_filter_5/dmavg_flt ==
  input : Inport
  omega : Inport  Port=2
  Compare To Zero : simulink/Logic and Bit Operations/Compare To Zero  relop=>  OutDataTypeStr=boolean
  Constant : Constant  Value=ts
  Enabled Subsystem : Subsystem  TreatAsAtomicUnit=on
  Step : Step  Time=enable_time
  Zero-Order Hold{,1..3} (4 alike) : ZeroOrderHold  SampleTime=-1
  dmavgflt_process : MATLAB Function  TreatAsAtomicUnit=on
  output : Outport
  wires:
  Zero-Order Hold3/1 -> dmavgflt_process/4(enable)
  Step/1 -> Zero-Order Hold3/1
  Zero-Order Hold1/1 -> dmavgflt_process/2(period)
  Zero-Order Hold2/1 -> dmavgflt_process/3(ts)
  Constant/1 -> Zero-Order Hold2/1
  Enabled Subsystem/1(Out1) -> Zero-Order Hold1/1
  Zero-Order Hold/1 -> dmavgflt_process/1(input)
  input/1 -> Zero-Order Hold/1
  omega/1 -> Enabled Subsystem/1(period), Compare To Zero/1
  Compare To Zero/1 -> Enabled Subsystem/Enable
  dmavgflt_process/1(output) -> output/1

== system three_phase_power_meter_iec/three_phase_power_meter_iec/iabc_sin_cos/simple_moving_average_filter_6/dmavg_flt ==
  input : Inport
  omega : Inport  Port=2
  Compare To Zero : simulink/Logic and Bit Operations/Compare To Zero  relop=>  OutDataTypeStr=boolean
  Constant : Constant  Value=ts
  Enabled Subsystem : Subsystem  TreatAsAtomicUnit=on
  Step : Step  Time=enable_time
  Zero-Order Hold{,1..3} (4 alike) : ZeroOrderHold  SampleTime=-1
  dmavgflt_process : MATLAB Function  TreatAsAtomicUnit=on
  output : Outport
  wires:
  dmavgflt_process/1(output) -> output/1
  Compare To Zero/1 -> Enabled Subsystem/Enable
  omega/1 -> Compare To Zero/1, Enabled Subsystem/1(period)
  input/1 -> Zero-Order Hold/1
  Zero-Order Hold/1 -> dmavgflt_process/1(input)
  Enabled Subsystem/1(Out1) -> Zero-Order Hold1/1
  Constant/1 -> Zero-Order Hold2/1
  Zero-Order Hold2/1 -> dmavgflt_process/3(ts)
  Zero-Order Hold1/1 -> dmavgflt_process/2(period)
  Step/1 -> Zero-Order Hold3/1
  Zero-Order Hold3/1 -> dmavgflt_process/4(enable)

== system three_phase_power_meter_iec/three_phase_power_meter_iec/uabc_sin_cos/simple_moving_average_filter_1/dmavg_flt ==
  input : Inport
  omega : Inport  Port=2
  Compare To Zero : simulink/Logic and Bit Operations/Compare To Zero  relop=>  OutDataTypeStr=boolean
  Constant : Constant  Value=ts
  Enabled Subsystem : Subsystem  TreatAsAtomicUnit=on
  Step : Step  Time=enable_time
  Zero-Order Hold{,1..3} (4 alike) : ZeroOrderHold  SampleTime=-1
  dmavgflt_process : MATLAB Function  TreatAsAtomicUnit=on
  output : Outport
  wires:
  Zero-Order Hold3/1 -> dmavgflt_process/4(enable)
  Step/1 -> Zero-Order Hold3/1
  Zero-Order Hold1/1 -> dmavgflt_process/2(period)
  Zero-Order Hold2/1 -> dmavgflt_process/3(ts)
  Constant/1 -> Zero-Order Hold2/1
  Enabled Subsystem/1(Out1) -> Zero-Order Hold1/1
  Zero-Order Hold/1 -> dmavgflt_process/1(input)
  input/1 -> Zero-Order Hold/1
  omega/1 -> Enabled Subsystem/1(period), Compare To Zero/1
  Compare To Zero/1 -> Enabled Subsystem/Enable
  dmavgflt_process/1(output) -> output/1

== system three_phase_power_meter_iec/three_phase_power_meter_iec/uabc_sin_cos/simple_moving_average_filter_2/dmavg_flt ==
  input : Inport
  omega : Inport  Port=2
  Compare To Zero : simulink/Logic and Bit Operations/Compare To Zero  relop=>  OutDataTypeStr=boolean
  Constant : Constant  Value=ts
  Enabled Subsystem : Subsystem  TreatAsAtomicUnit=on
  Step : Step  Time=enable_time
  Zero-Order Hold{,1..3} (4 alike) : ZeroOrderHold  SampleTime=-1
  dmavgflt_process : MATLAB Function  TreatAsAtomicUnit=on
  output : Outport
  wires:
  dmavgflt_process/1(output) -> output/1
  Compare To Zero/1 -> Enabled Subsystem/Enable
  omega/1 -> Compare To Zero/1, Enabled Subsystem/1(period)
  input/1 -> Zero-Order Hold/1
  Zero-Order Hold/1 -> dmavgflt_process/1(input)
  Enabled Subsystem/1(Out1) -> Zero-Order Hold1/1
  Constant/1 -> Zero-Order Hold2/1
  Zero-Order Hold2/1 -> dmavgflt_process/3(ts)
  Zero-Order Hold1/1 -> dmavgflt_process/2(period)
  Step/1 -> Zero-Order Hold3/1
  Zero-Order Hold3/1 -> dmavgflt_process/4(enable)

== system three_phase_power_meter_iec/three_phase_power_meter_iec/uabc_sin_cos/simple_moving_average_filter_3/dmavg_flt ==
  input : Inport
  omega : Inport  Port=2
  Compare To Zero : simulink/Logic and Bit Operations/Compare To Zero  relop=>  OutDataTypeStr=boolean
  Constant : Constant  Value=ts
  Enabled Subsystem : Subsystem  TreatAsAtomicUnit=on
  Step : Step  Time=enable_time
  Zero-Order Hold{,1..3} (4 alike) : ZeroOrderHold  SampleTime=-1
  dmavgflt_process : MATLAB Function  TreatAsAtomicUnit=on
  output : Outport
  wires:
  Zero-Order Hold3/1 -> dmavgflt_process/4(enable)
  Step/1 -> Zero-Order Hold3/1
  Zero-Order Hold1/1 -> dmavgflt_process/2(period)
  Zero-Order Hold2/1 -> dmavgflt_process/3(ts)
  Constant/1 -> Zero-Order Hold2/1
  Enabled Subsystem/1(Out1) -> Zero-Order Hold1/1
  Zero-Order Hold/1 -> dmavgflt_process/1(input)
  input/1 -> Zero-Order Hold/1
  omega/1 -> Enabled Subsystem/1(period), Compare To Zero/1
  Compare To Zero/1 -> Enabled Subsystem/Enable
  dmavgflt_process/1(output) -> output/1

== system three_phase_power_meter_iec/three_phase_power_meter_iec/uabc_sin_cos/simple_moving_average_filter_4/dmavg_flt ==
  input : Inport
  omega : Inport  Port=2
  Compare To Zero : simulink/Logic and Bit Operations/Compare To Zero  relop=>  OutDataTypeStr=boolean
  Constant : Constant  Value=ts
  Enabled Subsystem : Subsystem  TreatAsAtomicUnit=on
  Step : Step  Time=enable_time
  Zero-Order Hold{,1..3} (4 alike) : ZeroOrderHold  SampleTime=-1
  dmavgflt_process : MATLAB Function  TreatAsAtomicUnit=on
  output : Outport
  wires:
  dmavgflt_process/1(output) -> output/1
  Compare To Zero/1 -> Enabled Subsystem/Enable
  omega/1 -> Compare To Zero/1, Enabled Subsystem/1(period)
  input/1 -> Zero-Order Hold/1
  Zero-Order Hold/1 -> dmavgflt_process/1(input)
  Enabled Subsystem/1(Out1) -> Zero-Order Hold1/1
  Constant/1 -> Zero-Order Hold2/1
  Zero-Order Hold2/1 -> dmavgflt_process/3(ts)
  Zero-Order Hold1/1 -> dmavgflt_process/2(period)
  Step/1 -> Zero-Order Hold3/1
  Zero-Order Hold3/1 -> dmavgflt_process/4(enable)

== system three_phase_power_meter_iec/three_phase_power_meter_iec/uabc_sin_cos/simple_moving_average_filter_5/dmavg_flt ==
  input : Inport
  omega : Inport  Port=2
  Compare To Zero : simulink/Logic and Bit Operations/Compare To Zero  relop=>  OutDataTypeStr=boolean
  Constant : Constant  Value=ts
  Enabled Subsystem : Subsystem  TreatAsAtomicUnit=on
  Step : Step  Time=enable_time
  Zero-Order Hold{,1..3} (4 alike) : ZeroOrderHold  SampleTime=-1
  dmavgflt_process : MATLAB Function  TreatAsAtomicUnit=on
  output : Outport
  wires:
  Zero-Order Hold3/1 -> dmavgflt_process/4(enable)
  Step/1 -> Zero-Order Hold3/1
  Zero-Order Hold1/1 -> dmavgflt_process/2(period)
  Zero-Order Hold2/1 -> dmavgflt_process/3(ts)
  Constant/1 -> Zero-Order Hold2/1
  Enabled Subsystem/1(Out1) -> Zero-Order Hold1/1
  Zero-Order Hold/1 -> dmavgflt_process/1(input)
  input/1 -> Zero-Order Hold/1
  omega/1 -> Enabled Subsystem/1(period), Compare To Zero/1
  Compare To Zero/1 -> Enabled Subsystem/Enable
  dmavgflt_process/1(output) -> output/1

== system three_phase_power_meter_iec/three_phase_power_meter_iec/uabc_sin_cos/simple_moving_average_filter_6/dmavg_flt ==
  input : Inport
  omega : Inport  Port=2
  Compare To Zero : simulink/Logic and Bit Operations/Compare To Zero  relop=>  OutDataTypeStr=boolean
  Constant : Constant  Value=ts
  Enabled Subsystem : Subsystem  TreatAsAtomicUnit=on
  Step : Step  Time=enable_time
  Zero-Order Hold{,1..3} (4 alike) : ZeroOrderHold  SampleTime=-1
  dmavgflt_process : MATLAB Function  TreatAsAtomicUnit=on
  output : Outport
  wires:
  dmavgflt_process/1(output) -> output/1
  Compare To Zero/1 -> Enabled Subsystem/Enable
  omega/1 -> Compare To Zero/1, Enabled Subsystem/1(period)
  input/1 -> Zero-Order Hold/1
  Zero-Order Hold/1 -> dmavgflt_process/1(input)
  Enabled Subsystem/1(Out1) -> Zero-Order Hold1/1
  Constant/1 -> Zero-Order Hold2/1
  Zero-Order Hold2/1 -> dmavgflt_process/3(ts)
  Zero-Order Hold1/1 -> dmavgflt_process/2(period)
  Step/1 -> Zero-Order Hold3/1
  Zero-Order Hold3/1 -> dmavgflt_process/4(enable)

== system three_phase_power_meter_iec/three_phase_power_meter_iec/iabc_sin_cos/simple_moving_average_filter_1/dmavg_flt/Enabled Subsystem ==
  period : Inport
  Enable : EnablePort
  Constant2 : Constant
  Divide : Product  Inputs=*/
  Gain1 : Gain  Gain=1/(2*pi)
  Out1 : Outport
  wires:
  Divide/1 -> Out1/1  "period"
  Gain1/1 -> Divide/2
  period/1 -> Gain1/1  "omega"
  Constant2/1 -> Divide/1

== system three_phase_power_meter_iec/three_phase_power_meter_iec/iabc_sin_cos/simple_moving_average_filter_2/dmavg_flt/Enabled Subsystem ==
  period : Inport
  Enable : EnablePort
  Constant2 : Constant
  Divide : Product  Inputs=*/
  Gain1 : Gain  Gain=1/(2*pi)
  Out1 : Outport
  wires:
  Constant2/1 -> Divide/1
  period/1 -> Gain1/1  "omega"
  Gain1/1 -> Divide/2
  Divide/1 -> Out1/1  "period"

== system three_phase_power_meter_iec/three_phase_power_meter_iec/iabc_sin_cos/simple_moving_average_filter_3/dmavg_flt/Enabled Subsystem ==
  period : Inport
  Enable : EnablePort
  Constant2 : Constant
  Divide : Product  Inputs=*/
  Gain1 : Gain  Gain=1/(2*pi)
  Out1 : Outport
  wires:
  Divide/1 -> Out1/1  "period"
  Gain1/1 -> Divide/2
  period/1 -> Gain1/1  "omega"
  Constant2/1 -> Divide/1

== system three_phase_power_meter_iec/three_phase_power_meter_iec/iabc_sin_cos/simple_moving_average_filter_4/dmavg_flt/Enabled Subsystem ==
  period : Inport
  Enable : EnablePort
  Constant2 : Constant
  Divide : Product  Inputs=*/
  Gain1 : Gain  Gain=1/(2*pi)
  Out1 : Outport
  wires:
  Constant2/1 -> Divide/1
  period/1 -> Gain1/1  "omega"
  Gain1/1 -> Divide/2
  Divide/1 -> Out1/1  "period"

== system three_phase_power_meter_iec/three_phase_power_meter_iec/iabc_sin_cos/simple_moving_average_filter_5/dmavg_flt/Enabled Subsystem ==
  period : Inport
  Enable : EnablePort
  Constant2 : Constant
  Divide : Product  Inputs=*/
  Gain1 : Gain  Gain=1/(2*pi)
  Out1 : Outport
  wires:
  Divide/1 -> Out1/1  "period"
  Gain1/1 -> Divide/2
  period/1 -> Gain1/1  "omega"
  Constant2/1 -> Divide/1

== system three_phase_power_meter_iec/three_phase_power_meter_iec/iabc_sin_cos/simple_moving_average_filter_6/dmavg_flt/Enabled Subsystem ==
  period : Inport
  Enable : EnablePort
  Constant2 : Constant
  Divide : Product  Inputs=*/
  Gain1 : Gain  Gain=1/(2*pi)
  Out1 : Outport
  wires:
  Constant2/1 -> Divide/1
  period/1 -> Gain1/1  "omega"
  Gain1/1 -> Divide/2
  Divide/1 -> Out1/1  "period"

== system three_phase_power_meter_iec/three_phase_power_meter_iec/uabc_sin_cos/simple_moving_average_filter_1/dmavg_flt/Enabled Subsystem ==
  period : Inport
  Enable : EnablePort
  Constant2 : Constant
  Divide : Product  Inputs=*/
  Gain1 : Gain  Gain=1/(2*pi)
  Out1 : Outport
  wires:
  Divide/1 -> Out1/1  "period"
  Gain1/1 -> Divide/2
  period/1 -> Gain1/1  "omega"
  Constant2/1 -> Divide/1

== system three_phase_power_meter_iec/three_phase_power_meter_iec/uabc_sin_cos/simple_moving_average_filter_2/dmavg_flt/Enabled Subsystem ==
  period : Inport
  Enable : EnablePort
  Constant2 : Constant
  Divide : Product  Inputs=*/
  Gain1 : Gain  Gain=1/(2*pi)
  Out1 : Outport
  wires:
  Constant2/1 -> Divide/1
  period/1 -> Gain1/1  "omega"
  Gain1/1 -> Divide/2
  Divide/1 -> Out1/1  "period"

== system three_phase_power_meter_iec/three_phase_power_meter_iec/uabc_sin_cos/simple_moving_average_filter_3/dmavg_flt/Enabled Subsystem ==
  period : Inport
  Enable : EnablePort
  Constant2 : Constant
  Divide : Product  Inputs=*/
  Gain1 : Gain  Gain=1/(2*pi)
  Out1 : Outport
  wires:
  Divide/1 -> Out1/1  "period"
  Gain1/1 -> Divide/2
  period/1 -> Gain1/1  "omega"
  Constant2/1 -> Divide/1

== system three_phase_power_meter_iec/three_phase_power_meter_iec/uabc_sin_cos/simple_moving_average_filter_4/dmavg_flt/Enabled Subsystem ==
  period : Inport
  Enable : EnablePort
  Constant2 : Constant
  Divide : Product  Inputs=*/
  Gain1 : Gain  Gain=1/(2*pi)
  Out1 : Outport
  wires:
  Constant2/1 -> Divide/1
  period/1 -> Gain1/1  "omega"
  Gain1/1 -> Divide/2
  Divide/1 -> Out1/1  "period"

== system three_phase_power_meter_iec/three_phase_power_meter_iec/uabc_sin_cos/simple_moving_average_filter_5/dmavg_flt/Enabled Subsystem ==
  period : Inport
  Enable : EnablePort
  Constant2 : Constant
  Divide : Product  Inputs=*/
  Gain1 : Gain  Gain=1/(2*pi)
  Out1 : Outport
  wires:
  Divide/1 -> Out1/1  "period"
  Gain1/1 -> Divide/2
  period/1 -> Gain1/1  "omega"
  Constant2/1 -> Divide/1

== system three_phase_power_meter_iec/three_phase_power_meter_iec/uabc_sin_cos/simple_moving_average_filter_6/dmavg_flt/Enabled Subsystem ==
  period : Inport
  Enable : EnablePort
  Constant2 : Constant
  Divide : Product  Inputs=*/
  Gain1 : Gain  Gain=1/(2*pi)
  Out1 : Outport
  wires:
  Constant2/1 -> Divide/1
  period/1 -> Gain1/1  "omega"
  Gain1/1 -> Divide/2
  Divide/1 -> Out1/1  "period"

== matlab function three_phase_power_meter_iec/uabc_sin_cos/simple_moving_average_filter_3/dmavg_flt/dmavgflt_process ==
  data: input input; output output; period input; ts input; enable input
function output = dmavgflt_process(input, period, ts, enable)
%#codegen
% DMAVGFLT_PROCESS  Dynamic Moving Average Filter con periodo variabile e frazionario
%
%   output = dmavgflt_process(input, period, ts)
%
%   Filtro a media mobile con:
%   - Buffer circolare
%   - Periodo variabile e frazionario
%   - Aggiornamento incrementale (alta efficienza)
%
%   Compatibile con Simulink (persistent variables)
%   ts (s) : sampling time
%   period (s) : periodo su cui si vuole fare la media
%   input : segnale da mediare.

    % Parametri fissi
    MAVGFLT_SIZE_MAX = 17500; % MAVGFLT_SIZE_MAX > di 200ms/125us

    % Variabili persistenti (mantengono lo stato tra chiamate)
    persistent buffer cb_index sample_count sum_short sum_long prev_input

    % Inizializzazione al primo passo
    if isempty(buffer)
        buffer       = zeros(1, MAVGFLT_SIZE_MAX); %vettore del buffer circolare (1×MAVGFLT_SIZE_MAX)
        cb_index     = 1;   % current buffer index: indice di scrittura corrente
        sample_count = 1;   % sample count : numero di campioni attivi nella finestra, questo
                            % (e il suo sample_count-1) è il numero di
                            % campioni con cui farò la media.
                            % sample_count parte da zero e man mano cresce
                            % e viene aumentato e contratto a seconda del
                            % valore di n_samples.
        sum_short    = 0;   % somma corta
        sum_long     = 0;   % somma lunga
        prev_input   = 0;   % ultimo valore di ingresso 
    end

    if enable 
        % Gestione caso periodo nullo o negativo
        if period <= 0
            output = 0;
            return;
        end
    
        % Numero desiderato di campioni: è un nemero reale
        desired_samples = period / ts;
    
        % Limite massimo
        if desired_samples > (MAVGFLT_SIZE_MAX - 1)
            desired_samples = MAVGFLT_SIZE_MAX - 1;
        end
    
        % Parte intera e frazionaria
        % es: 
        % desired_samples = 20.8
        % n_samples = 21
        % frac = 0.8
        % desired_samples = 20.2
        % n_samples = 21
        % frac = 0.2

        % numero di campioni che coprono interamente il periodo
        n_samples = floor(desired_samples + 1); 
        % parte prazionaria 
        frac = desired_samples + 1 - n_samples; 
    
        % Evita finestre vuote
        if n_samples < 1
            n_samples = 1;
        end
    
        % Aggiornamento sample_count: sample_count verrà aumentato, 
        % calato o mantenuto costante a seconda della differenza fra 
        % n_samples.
        if n_samples > sample_count
            
            % Finestra aumenta → aggiungi nuovi campioni
            sum_short = sum_short + prev_input;
            sum_long  = sum_long  + input;
            
            sample_count = sample_count + 1;
    
        elseif n_samples < sample_count
            
            % Finestra ridotta → rimuovi i campioni più vecchi
            oldest_sample_idx1 = buffer_index(cb_index, sample_count, MAVGFLT_SIZE_MAX);
            oldest_sample_idx2 = buffer_index(cb_index, sample_count - 1, MAVGFLT_SIZE_MAX);
            oldest_sample_1 = buffer(oldest_sample_idx1);
            oldest_sample_2 = buffer(oldest_sample_idx2);
            oldest_samples_sum = oldest_sample_1 + oldest_sample_2;
    
            sum_short = sum_short + prev_input - oldest_samples_sum;
            sum_long  = sum_long  + input - oldest_samples_sum;
    
            sample_count = sample_count - 1;
    
        else
            % Finestra costante
            oldest_sample = buffer_value(buffer, cb_index, sample_count, MAVGFLT_SIZE_MAX);
            sum_short = sum_short + prev_input - oldest_sample;
            sum_long  = sum_long  + input - oldest_sample;
        end
    
        % --- Aggiornamento buffer circolare ---
        buffer(cb_index) = input;
        cb_index = mod(cb_index, MAVGFLT_SIZE_MAX) + 1;
        prev_input = input;
    
        % --- Calcolo output ---
        if sample_count > 1
            avg_short = sum_short / (sample_count - 1);
        else
            avg_short = 0;
        end
        avg_long = sum_long / sample_count;
    
        % Interpolazione lineare tra finestre
        output = avg_short * (1 - frac) + avg_long * frac;
    else
        output = 0;
    end
end


% funzioni gestion buffer circolare
function idx = buffer_index(cb_index, offset, max_size)
% Calcola indice 1-based di un campione "offset" passi indietro nel buffer
% circolare
    idx = mod(cb_index - 1 - offset, max_size) + 1;
end

function val = buffer_value(buffer, cb_index, offset, max_size)
% Restituisce il valore del buffer "offset" passi indietro
    idx = mod(cb_index - 1 - offset, max_size) + 1;
    val = buffer(idx);
end

== matlab function three_phase_power_meter_iec/uabc_sin_cos/simple_moving_average_filter_4/dmavg_flt/dmavgflt_process ==
  data: input input; output output; period input; ts input; enable input
function output = dmavgflt_process(input, period, ts, enable)
%#codegen
% DMAVGFLT_PROCESS  Dynamic Moving Average Filter con periodo variabile e frazionario
%
%   output = dmavgflt_process(input, period, ts)
%
%   Filtro a media mobile con:
%   - Buffer circolare
%   - Periodo variabile e frazionario
%   - Aggiornamento incrementale (alta efficienza)
%
%   Compatibile con Simulink (persistent variables)
%   ts (s) : sampling time
%   period (s) : periodo su cui si vuole fare la media
%   input : segnale da mediare.

    % Parametri fissi
    MAVGFLT_SIZE_MAX = 17500; % MAVGFLT_SIZE_MAX > di 200ms/125us

    % Variabili persistenti (mantengono lo stato tra chiamate)
    persistent buffer cb_index sample_count sum_short sum_long prev_input

    % Inizializzazione al primo passo
    if isempty(buffer)
        buffer       = zeros(1, MAVGFLT_SIZE_MAX); %vettore del buffer circolare (1×MAVGFLT_SIZE_MAX)
        cb_index     = 1;   % current buffer index: indice di scrittura corrente
        sample_count = 1;   % sample count : numero di campioni attivi nella finestra, questo
                            % (e il suo sample_count-1) è il numero di
                            % campioni con cui farò la media.
                            % sample_count parte da zero e man mano cresce
                            % e viene aumentato e contratto a seconda del
                            % valore di n_samples.
        sum_short    = 0;   % somma corta
        sum_long     = 0;   % somma lunga
        prev_input   = 0;   % ultimo valore di ingresso 
    end

    if enable 
        % Gestione caso periodo nullo o negativo
        if period <= 0
            output = 0;
            return;
        end
    
        % Numero desiderato di campioni: è un nemero reale
        desired_samples = period / ts;
    
        % Limite massimo
        if desired_samples > (MAVGFLT_SIZE_MAX - 1)
            desired_samples = MAVGFLT_SIZE_MAX - 1;
        end
    
        % Parte intera e frazionaria
        % es: 
        % desired_samples = 20.8
        % n_samples = 21
        % frac = 0.8
        % desired_samples = 20.2
        % n_samples = 21
        % frac = 0.2

        % numero di campioni che coprono interamente il periodo
        n_samples = floor(desired_samples + 1); 
        % parte prazionaria 
        frac = desired_samples + 1 - n_samples; 
    
        % Evita finestre vuote
        if n_samples < 1
            n_samples = 1;
        end
    
        % Aggiornamento sample_count: sample_count verrà aumentato, 
        % calato o mantenuto costante a seconda della differenza fra 
        % n_samples.
        if n_samples > sample_count
            
            % Finestra aumenta → aggiungi nuovi campioni
            sum_short = sum_short + prev_input;
            sum_long  = sum_long  + input;
            
            sample_count = sample_count + 1;
    
        elseif n_samples < sample_count
            
            % Finestra ridotta → rimuovi i campioni più vecchi
            oldest_sample_idx1 = buffer_index(cb_index, sample_count, MAVGFLT_SIZE_MAX);
            oldest_sample_idx2 = buffer_index(cb_index, sample_count - 1, MAVGFLT_SIZE_MAX);
            oldest_sample_1 = buffer(oldest_sample_idx1);
            oldest_sample_2 = buffer(oldest_sample_idx2);
            oldest_samples_sum = oldest_sample_1 + oldest_sample_2;
    
            sum_short = sum_short + prev_input - oldest_samples_sum;
            sum_long  = sum_long  + input - oldest_samples_sum;
    
            sample_count = sample_count - 1;
    
        else
            % Finestra costante
            oldest_sample = buffer_value(buffer, cb_index, sample_count, MAVGFLT_SIZE_MAX);
            sum_short = sum_short + prev_input - oldest_sample;
            sum_long  = sum_long  + input - oldest_sample;
        end
    
        % --- Aggiornamento buffer circolare ---
        buffer(cb_index) = input;
        cb_index = mod(cb_index, MAVGFLT_SIZE_MAX) + 1;
        prev_input = input;
    
        % --- Calcolo output ---
        if sample_count > 1
            avg_short = sum_short / (sample_count - 1);
        else
            avg_short = 0;
        end
        avg_long = sum_long / sample_count;
    
        % Interpolazione lineare tra finestre
        output = avg_short * (1 - frac) + avg_long * frac;
    else
        output = 0;
    end
end


% funzioni gestion buffer circolare
function idx = buffer_index(cb_index, offset, max_size)
% Calcola indice 1-based di un campione "offset" passi indietro nel buffer
% circolare
    idx = mod(cb_index - 1 - offset, max_size) + 1;
end

function val = buffer_value(buffer, cb_index, offset, max_size)
% Restituisce il valore del buffer "offset" passi indietro
    idx = mod(cb_index - 1 - offset, max_size) + 1;
    val = buffer(idx);
end
